simulink model "ur5_pid"  (R2026b)
settings: Solver=ode45  StopTime=Tend  MaxStep=1e-3  RelTol=1e-5
undefined symbols (not defined in the file): KdP, KiP, KpP, NB, q0, sigmaQ, sigmaQd, tauMax
libraries: robotmaniplib x1
settings Model: Creator=har  LastModifiedBy=har

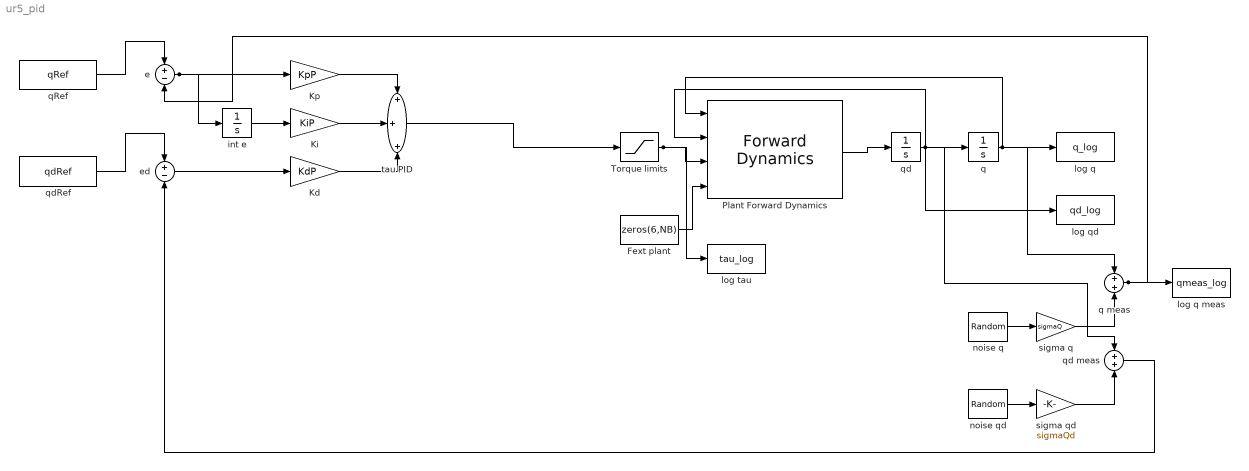
== system ur5_pid ==
  Fext plant : Constant  Value=zeros(6,NB)
  Kd : Gain  Gain=KdP
  Ki : Gain  Gain=KiP
  Kp : Gain  Gain=KpP
  Plant Forward Dynamics : robotmaniplib/Forward Dynamics  RigidBodyTree=robotPlant  SimulateUsing=Code generation
  Torque limits : Saturate  UpperLimit=tauMax  LowerLimit=-tauMax
  e : Sum  Inputs=+-
  ed : Sum  Inputs=+-
  int e : Integrator  InitialCondition=zeros(6,1)
  log q : ToWorkspace  VariableName=q_log  SaveFormat=Timeseries  SampleTime=-1
  log q meas : ToWorkspace  VariableName=qmeas_log  SaveFormat=Timeseries  SampleTime=-1
  log qd : ToWorkspace  VariableName=qd_log  SaveFormat=Timeseries  SampleTime=-1
  log tau : ToWorkspace  VariableName=tau_log  SaveFormat=Timeseries  SampleTime=-1
  noise q : RandomNumber  Mean=zeros(6,1)  Variance=ones(6,1)  Seed=[11 12 13 14 15 16]  SampleTime=1e-3
  noise qd : RandomNumber  Mean=zeros(6,1)  Variance=ones(6,1)  Seed=[21 22 23 24 25 26]  SampleTime=1e-3
  q : Integrator  InitialCondition=q0
  q meas : Sum
  qRef : FromWorkspace  VariableName=qRef  OutputAfterFinalValue=Holding final value
  qd : Integrator  InitialCondition=zeros(6,1)
  qd meas : Sum
  qdRef : FromWorkspace  VariableName=qdRef  OutputAfterFinalValue=Holding final value
  sigma q : Gain  Gain=sigmaQ
  sigma qd : Gain  Gain=sigmaQd
  tau PID : Sum  Inputs=+++
  wires:
  q/1 -> q meas/1, Plant Forward Dynamics/1, log q/1
  noise q/1 -> sigma q/1
  sigma q/1 -> q meas/2
  qd/1 -> qd meas/1, Plant Forward Dynamics/2, q/1, log qd/1
  noise qd/1 -> sigma qd/1
  sigma qd/1 -> qd meas/2
  qRef/1 -> e/1
  q meas/1 -> e/2, log q meas/1
  qdRef/1 -> ed/1
  qd meas/1 -> ed/2
  e/1 -> int e/1, Kp/1
  int e/1 -> Ki/1
  ed/1 -> Kd/1
  Kp/1 -> tau PID/1
  Ki/1 -> tau PID/2
  Kd/1 -> tau PID/3
  tau PID/1 -> Torque limits/1
  Torque limits/1 -> Plant Forward Dynamics/3, log tau/1
  Fext plant/1 -> Plant Forward Dynamics/4
  Plant Forward Dynamics/1 -> qd/1
